simulink model "DCMachine"  (R2025b)
settings: Solver=FixedStepAuto  StartTime=0.0  StopTime=2000  FixedStep=0.01  RelTol=1e-3
values from neighbouring files (symbols this model uses):
  beta = 0.81    [DC_Motor3.m]
  d = 0.68    [DC_Motor3.m]
  En = 600-Ra*156    (= 539.16)    [DC_Motor3.m]
  I_en = 5    [DC_Motor3.m]
  Ia_max = 156    [DC_Motor3.m]
  Jeq = m_total * (rho^2 * d^2) / 4    (= 90.6180715851)    [DC_Motor3.m]
  Ki_a = Ca.Ki    [DC_Motor3.m]
  Ki_e = Ce.Ki    [DC_Motor3.m]
  Ki_w = Cw.Ki    [DC_Motor3.m]
  Kp_a = Ca.Kp    [DC_Motor3.m]
  Kp_e = Ce.Kp    [DC_Motor3.m]
  Kp_w = Cw.Kp    [DC_Motor3.m]
  Kt = 1.06    [DC_Motor3.m]
  La = tau_a * Ra    (= 0.0039)    [DC_Motor3.m]
  Le = tau_e * Re    (= 1.2)    [DC_Motor3.m]
  m_total = m_tram + m_passengers    (= 25400)    [DC_Motor3.m]
  Omega_b = 970 * (2*pi/60)    (= 101.578162466)    [DC_Motor3.m]
  Ra = 0.39    [DC_Motor3.m]
  Re = 12    [DC_Motor3.m]
  rho = 13/74    (= 0.175675675676)    [DC_Motor3.m]
  V_max = 42 * 1000/3600    (= 11.6666666667)    [DC_Motor3.m]
  V_r = Omega_b * rho * d/2    (= 6.06723619054)    [DC_Motor3.m]
libraries: slpidlib x3, simulink x1
settings Model: Creator=ASUS  LastModifiedBy=sanaz

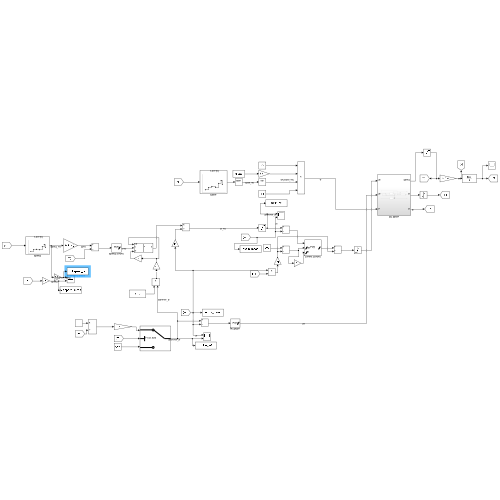
[thumbnail: Simulink's stored preview of the top-level diagram]
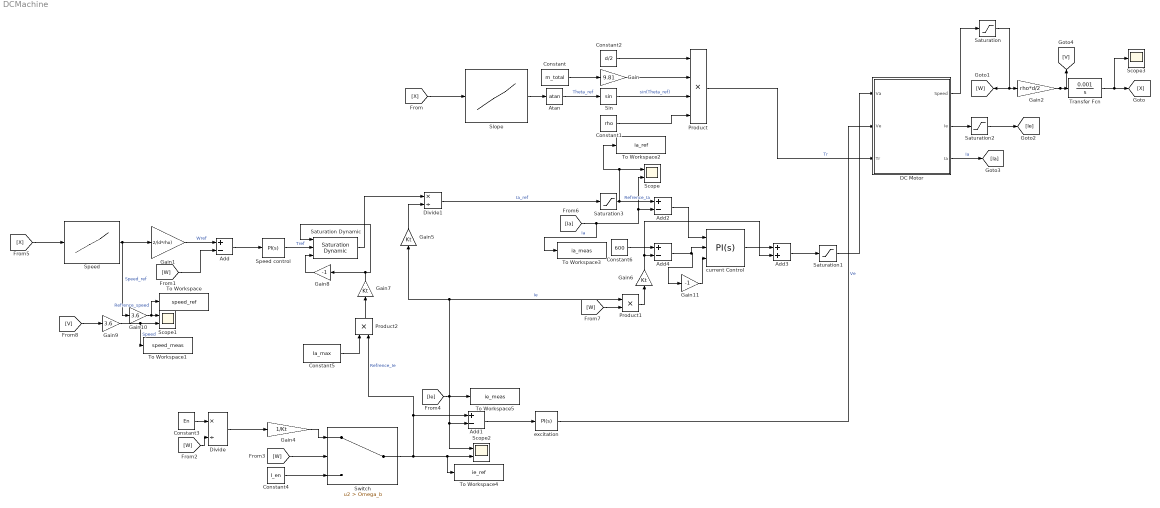
== system DCMachine ==
  Add{,1..2,4} (4 alike) : Sum  Inputs=+-
  Add3 : Sum
  Atan : Trigonometry  Operator=atan
  Constant : Constant  Value=m_total
  Constant1 : Constant  Value=rho
  Constant2 : Constant  Value=d/2
  Constant3 : Constant  Value=En
  Constant4 : Constant  Value=I_en
  Constant5 : Constant  Value=Ia_max
  Constant6 : Constant  Value=600
  DC Motor : Subsystem
  Divide : Product  Inputs=*/
  Divide1 : Product  Inputs=*/
  Gain : Gain  Gain=9.81
  Gain1 : Gain  Gain=2/(d*rho)
  Gain10 : Gain  Gain=3.6
  Gain11 : Gain  Gain=-1
  Gain2 : Gain  Gain=rho*d/2
  Gain4 : Gain  Gain=1/Kt
  Gain5 : Gain  Gain=Kt
  Gain6 : Gain  Gain=Kt
  Gain7 : Gain  Gain=Kt
  Gain8 : Gain  Gain=-1
  Gain9 : Gain  Gain=3.6
  Product : Product  Inputs=4
  Product1 : Product
  Product2 : Product
  Saturation : Saturate  UpperLimit=V_max/ (rho*d/2)  LowerLimit=-V_max/ (rho*d/2)
  Saturation Dynamic : simulink/Discontinuities/Saturation Dynamic  OutMin=[]  OutMax=[]  OutDataTypeStr=Inherit: Same as second input  OutDataType=fixdt(1, 16)  OutScaling=2^-10  DoSatur=off
  Saturation1 : Saturate  UpperLimit=600  LowerLimit=-600
  Saturation2 : Saturate  UpperLimit=inf  LowerLimit=0.0001
  Saturation3 : Saturate  UpperLimit=156  LowerLimit=-156
  Scope : Scope  NumInputPorts=2
      settings: ActiveDisplayYMinimum=-728.14495433164473  ActiveDisplayYMaximum=771.63756119337165
  Scope1 : Scope  NumInputPorts=2
      settings: ActiveDisplayYMinimum=-24.946598374660528  ActiveDisplayYMaximum=27.001405969121826
  Scope2 : Scope  NumInputPorts=2
      settings: ActiveDisplayYMinimum=-1.1065409547729188  ActiveDisplayYMaximum=6.7298853808900017  DataLoggingVariableName=ScopeData2
  Scope3 : Scope
      settings: ActiveDisplayYMinimum=-2.2097734184935658  ActiveDisplayYMaximum=19.887960766442095  DataLoggingVariableName=ScopeData3
  Sin : Trigonometry
  Slope : Lookup_n-D  NumberOfTableDimensions=1  LookupTableObject=''  BreakpointsForDimension1=[0, 1, 3, 4, 6, 8, 9, 10,10.1]  BreakpointsForDimension2=[1:2]  BreakpointsForDimension3=[5, 7]  BreakpointsForDimension1FirstPoint=10  BreakpointsForDimension2FirstPoint=10  BreakpointsForDimension1Spacing=12  BreakpointsForDimension2Spacing=12  Table=[0,0,0.05,0,0,-0.05,0,0,0]  InterpMethod=Flat  DiagnosticForOutOfRangeInput=Warning  InternalRulePriority=Speed  RndMeth=Simplest
  Speed : Lookup_n-D  NumberOfTableDimensions=1  BreakpointsForDimension1=[0, 1, 3, 4, 6, 8, 9, 10]  Table=[V_r/2,V_r,V_r,V_max,V_r,V_r,V_r/2,0]  InterpMethod=Flat  InternalRulePriority=Speed  RndMeth=Simplest
  Speed control : slpidlib/PID Controller  Controller=PI  Form=Parallel  TimeDomain=Continuous-time  UseExternalTs=off  SampleTime=-1  IntegratorMethod=Forward Euler  FilterMethod=Forward Euler  ControllerParametersSource=internal  P=Kp_w  I=Ki_w  UseKiTs=off  D=0  UseExternalDerivativeSource=off  N=100  UseFilter=on  TunerSelectOption=Transfer Function Based (PID Tuner App)  InitialConditionSource=internal  InitialConditionForIntegrator=0  InitialConditionForFilter=0  DifferentiatorICPrevScaledInput=0  ExternalReset=none  TrackingMode=off  Kt=1  LimitOutput=on  SatLimitsSource=internal  UpperSaturationLimit=827  LowerSaturationLimit=-827  LinearizeAsGain=on  AntiWindupMode=back-calculation  Kb=Ki_w/Kp_w  LimitIntegrator=on  UpperIntegratorSaturationLimit=inf  LowerIntegratorSaturationLimit=-inf  POutMin=[]  POutMax=[]  IOutMin=[]  IOutMax=[]  DOutMin=[]  DOutMax=[]  NOutMin=[]  NOutMax=[]  SumOutMin=[]  SumOutMax=[]  SaturationOutMin=[]  SaturationOutMax=[]  PParamMin=[]  PParamMax=[]  IParamMin=[]  IParamMax=[]  DParamMin=[]  DParamMax=[]  NParamMin=[]  NParamMax=[]  KbParamMin=[]  KbParamMax=[]  KtParamMin=[]  KtParamMax=[]  KbOutMin=[]  KbOutMax=[]  KtOutMin=[]  KtOutMax=[]  IntegratorOutMin=[]  IntegratorOutMax=[]  FilterOutMin=[]  FilterOutMax=[]  SumI1OutMin=[]  SumI1OutMax=[]  SumI2OutMin=[]  SumI2OutMax=[]  SumI3OutMin=[]  SumI3OutMax=[]  SumI4OutMin=[]  SumI4OutMax=[]  SumDOutMin=[]  SumDOutMax=[]  DifferentiatorOutMin=[]  DifferentiatorOutMax=[]  FilterDiffOutCoefMin=[]  FilterDiffOutCoefMax=[]  ReciprocalOutMin=[]  ReciprocalOutMax=[]  SumDenOutMin=[]  SumDenOutMax=[]  SumNumOutMin=[]  SumNumOutMax=[]  DivideOutMin=[]  DivideOutMax=[]  UdiffTsProdOutMin=[]  UdiffTsProdOutMax=[]  NTsProdOutMin=[]  NTsProdOutMax=[]  UintegralTsProdOutMin=[]  UintegralTsProdOutMax=[]  UngainTsProdOutMin=[]  UngainTsProdOutMax=[]  ClampingZeroOutDataTypeStr=Inherit: Inherit via back propagation  ClampingZeroOutMin=[]  ClampingZeroOutMax=[]  FilterDenConstantOutDataTypeStr=Inherit: Inherit via back propagation  FilterDenConstantOutMin=[]  FilterDenConstantOutMax=[]  PCopyOutDataTypeStr=Inherit: Inherit via back propagation  PCopyOutMin=[]  PCopyOutMax=[]  NCopyOutDataTypeStr=Inherit: Inherit via back propagation  NCopyOutMin=[]  NCopyOutMax=[]  IntegratorContinuousStateAttributes=''  IntegratorStateMustResolveToSignalObject=off  IntegratorRTWStateStorageClass=Auto  FilterContinuousStateAttributes=''  FilterStateMustResolveToSignalObject=off  FilterRTWStateStorageClass=Auto  ParallelPVariant=InternalParameters  IdealPVariant=Disabled  IVariant=InternalParameters  DVariant=Disabled  IntegratorVariant=Continuous  SatVariant=Enabled  AWVariant=BackCalculation  PCopyVariant=Disabled  TRVariant=Disabled  FdbkBlocksVariant=Forward  IdealPFdbkVariant=Disabled  SatFdbkVariant=Disabled  DerivativeFilterVariant=Disabled  NVariant=Disabled  NCopyVariant=Disabled_SignalSpec  FilterICVariant=Disabled  IntegratorICVariant=InternalICs  ExternalResetVariant=Disabled  TRSumVariant=Passthrough  SumFdbkVariant=Disabled  SumVariant=Sum_PI  TsampFilterVariant=InternalTs  TsampNgainVariant=Passthrough  TsampIntegralVariant=Disabled_SignalSpec  ExternalSaturationOutDataTypeStr=Inherit: Same as second input  DerivativeSourceVariant=Disabled  PreIntVariant=InternalPreInt
  Switch : Switch  Criteria=u2 > Threshold  Threshold=Omega_b  SaturateOnIntegerOverflow=off  InputSameDT=off
  To Workspace : ToWorkspace  VariableName=speed_ref  SaveFormat=Timeseries  SampleTime=-1
  To Workspace1 : ToWorkspace  VariableName=speed_meas  SaveFormat=Timeseries  SampleTime=-1
  To Workspace2 : ToWorkspace  VariableName=ia_ref  SaveFormat=Timeseries  SampleTime=-1
  To Workspace3 : ToWorkspace  VariableName=ia_meas  SaveFormat=Timeseries  SampleTime=-1
  To Workspace4 : ToWorkspace  VariableName=ie_ref  SaveFormat=Timeseries  SampleTime=-1
  To Workspace5 : ToWorkspace  VariableName=ie_meas  SaveFormat=Timeseries  SampleTime=-1
  Transfer Fcn : TransferFcn  Numerator=[0.001]  Denominator=[1 0]
  current Control : slpidlib/PID Controller  Controller=PI  Form=Parallel  TimeDomain=Continuous-time  UseExternalTs=off  SampleTime=-1  IntegratorMethod=Forward Euler  FilterMethod=Forward Euler  ControllerParametersSource=internal  P=Kp_a  I=Ki_a  UseKiTs=off  D=0  UseExternalDerivativeSource=off  N=100  UseFilter=on  TunerSelectOption=Transfer Function Based (PID Tuner App)  InitialConditionSource=internal  InitialConditionForIntegrator=0  InitialConditionForFilter=0  DifferentiatorICPrevScaledInput=0  ExternalReset=none  TrackingMode=off  Kt=1  LimitOutput=on  SatLimitsSource=external  UpperSaturationLimit=inf  LowerSaturationLimit=-inf  LinearizeAsGain=on  AntiWindupMode=back-calculation  Kb=Ki_a/Kp_a  LimitIntegrator=off  UpperIntegratorSaturationLimit=inf  LowerIntegratorSaturationLimit=-inf  POutMin=[]  POutMax=[]  IOutMin=[]  IOutMax=[]  DOutMin=[]  DOutMax=[]  NOutMin=[]  NOutMax=[]  SumOutMin=[]  SumOutMax=[]  SaturationOutMin=[]  SaturationOutMax=[]  PParamMin=[]  PParamMax=[]  IParamMin=[]  IParamMax=[]  DParamMin=[]  DParamMax=[]  NParamMin=[]  NParamMax=[]  KbParamMin=[]  KbParamMax=[]  KtParamMin=[]  KtParamMax=[]  KbOutMin=[]  KbOutMax=[]  KtOutMin=[]  KtOutMax=[]  IntegratorOutMin=[]  IntegratorOutMax=[]  FilterOutMin=[]  FilterOutMax=[]  SumI1OutMin=[]  SumI1OutMax=[]  SumI2OutMin=[]  SumI2OutMax=[]  SumI3OutMin=[]  SumI3OutMax=[]  SumI4OutMin=[]  SumI4OutMax=[]  SumDOutMin=[]  SumDOutMax=[]  DifferentiatorOutMin=[]  DifferentiatorOutMax=[]  FilterDiffOutCoefMin=[]  FilterDiffOutCoefMax=[]  ReciprocalOutMin=[]  ReciprocalOutMax=[]  SumDenOutMin=[]  SumDenOutMax=[]  SumNumOutMin=[]  SumNumOutMax=[]  DivideOutMin=[]  DivideOutMax=[]  UdiffTsProdOutMin=[]  UdiffTsProdOutMax=[]  NTsProdOutMin=[]  NTsProdOutMax=[]  UintegralTsProdOutMin=[]  UintegralTsProdOutMax=[]  UngainTsProdOutMin=[]  UngainTsProdOutMax=[]  ClampingZeroOutDataTypeStr=Inherit: Inherit via back propagation  ClampingZeroOutMin=[]  ClampingZeroOutMax=[]  FilterDenConstantOutDataTypeStr=Inherit: Inherit via back propagation  FilterDenConstantOutMin=[]  FilterDenConstantOutMax=[]  PCopyOutDataTypeStr=Inherit: Inherit via back propagation  PCopyOutMin=[]  PCopyOutMax=[]  NCopyOutDataTypeStr=Inherit: Inherit via back propagation  NCopyOutMin=[]  NCopyOutMax=[]  IntegratorContinuousStateAttributes=''  IntegratorStateMustResolveToSignalObject=off  IntegratorRTWStateStorageClass=Auto  FilterContinuousStateAttributes=''  FilterStateMustResolveToSignalObject=off  FilterRTWStateStorageClass=Auto  ParallelPVariant=InternalParameters  IdealPVariant=Disabled  IVariant=InternalParameters  DVariant=Disabled  IntegratorVariant=Continuous  SatVariant=External  AWVariant=BackCalculation  PCopyVariant=Disabled  TRVariant=Disabled  FdbkBlocksVariant=Forward  IdealPFdbkVariant=Disabled  SatFdbkVariant=Disabled  DerivativeFilterVariant=Disabled  NVariant=Disabled  NCopyVariant=Disabled_SignalSpec  FilterICVariant=Disabled  IntegratorICVariant=InternalICs  ExternalResetVariant=Disabled  TRSumVariant=Passthrough  SumFdbkVariant=Disabled  SumVariant=Sum_PI  TsampFilterVariant=InternalTs  TsampNgainVariant=Passthrough  TsampIntegralVariant=Disabled_SignalSpec  ExternalSaturationOutDataTypeStr=Inherit: Same as second input  DerivativeSourceVariant=Disabled  PreIntVariant=InternalPreInt
  excitation : slpidlib/PID Controller  Controller=PI  Form=Parallel  TimeDomain=Continuous-time  UseExternalTs=off  SampleTime=-1  IntegratorMethod=Forward Euler  FilterMethod=Forward Euler  ControllerParametersSource=internal  P=Kp_e  I=Ki_e  UseKiTs=off  D=0  UseExternalDerivativeSource=off  N=100  UseFilter=on  TunerSelectOption=Transfer Function Based (PID Tuner App)  InitialConditionSource=internal  InitialConditionForIntegrator=0  InitialConditionForFilter=0  DifferentiatorICPrevScaledInput=0  ExternalReset=none  TrackingMode=off  Kt=1  LimitOutput=on  SatLimitsSource=internal  UpperSaturationLimit=60  LowerSaturationLimit=0  LinearizeAsGain=on  AntiWindupMode=back-calculation  Kb=Ki_e/Kp_e  LimitIntegrator=off  UpperIntegratorSaturationLimit=inf  LowerIntegratorSaturationLimit=-inf  POutMin=[]  POutMax=[]  IOutMin=[]  IOutMax=[]  DOutMin=[]  DOutMax=[]  NOutMin=[]  NOutMax=[]  SumOutMin=[]  SumOutMax=[]  SaturationOutMin=[]  SaturationOutMax=[]  PParamMin=[]  PParamMax=[]  IParamMin=[]  IParamMax=[]  DParamMin=[]  DParamMax=[]  NParamMin=[]  NParamMax=[]  KbParamMin=[]  KbParamMax=[]  KtParamMin=[]  KtParamMax=[]  KbOutMin=[]  KbOutMax=[]  KtOutMin=[]  KtOutMax=[]  IntegratorOutMin=[]  IntegratorOutMax=[]  FilterOutMin=[]  FilterOutMax=[]  SumI1OutMin=[]  SumI1OutMax=[]  SumI2OutMin=[]  SumI2OutMax=[]  SumI3OutMin=[]  SumI3OutMax=[]  SumI4OutMin=[]  SumI4OutMax=[]  SumDOutMin=[]  SumDOutMax=[]  DifferentiatorOutMin=[]  DifferentiatorOutMax=[]  FilterDiffOutCoefMin=[]  FilterDiffOutCoefMax=[]  ReciprocalOutMin=[]  ReciprocalOutMax=[]  SumDenOutMin=[]  SumDenOutMax=[]  SumNumOutMin=[]  SumNumOutMax=[]  DivideOutMin=[]  DivideOutMax=[]  UdiffTsProdOutMin=[]  UdiffTsProdOutMax=[]  NTsProdOutMin=[]  NTsProdOutMax=[]  UintegralTsProdOutMin=[]  UintegralTsProdOutMax=[]  UngainTsProdOutMin=[]  UngainTsProdOutMax=[]  ClampingZeroOutDataTypeStr=Inherit: Inherit via back propagation  ClampingZeroOutMin=[]  ClampingZeroOutMax=[]  FilterDenConstantOutDataTypeStr=Inherit: Inherit via back propagation  FilterDenConstantOutMin=[]  FilterDenConstantOutMax=[]  PCopyOutDataTypeStr=Inherit: Inherit via back propagation  PCopyOutMin=[]  PCopyOutMax=[]  NCopyOutDataTypeStr=Inherit: Inherit via back propagation  NCopyOutMin=[]  NCopyOutMax=[]  IntegratorContinuousStateAttributes=''  IntegratorStateMustResolveToSignalObject=off  IntegratorRTWStateStorageClass=Auto  FilterContinuousStateAttributes=''  FilterStateMustResolveToSignalObject=off  FilterRTWStateStorageClass=Auto  ParallelPVariant=InternalParameters  IdealPVariant=Disabled  IVariant=InternalParameters  DVariant=Disabled  IntegratorVariant=Continuous  SatVariant=Enabled  AWVariant=BackCalculation  PCopyVariant=Disabled  TRVariant=Disabled  FdbkBlocksVariant=Forward  IdealPFdbkVariant=Disabled  SatFdbkVariant=Disabled  DerivativeFilterVariant=Disabled  NVariant=Disabled  NCopyVariant=Disabled_SignalSpec  FilterICVariant=Disabled  IntegratorICVariant=InternalICs  ExternalResetVariant=Disabled  TRSumVariant=Passthrough  SumFdbkVariant=Disabled  SumVariant=Sum_PI  TsampFilterVariant=InternalTs  TsampNgainVariant=Passthrough  TsampIntegralVariant=Disabled_SignalSpec  ExternalSaturationOutDataTypeStr=Inherit: Same as second input  DerivativeSourceVariant=Disabled  PreIntVariant=InternalPreInt
  wires:
  Slope/1 -> Atan/1
  Atan/1 -> Sin/1  "Theta_ref"
  Constant/1 -> Gain/1
  Gain/1 -> Product/2
  Sin/1 -> Product/3  "sin(Theta_ref)"
  Constant1/1 -> Product/4
  Speed/1 -> Gain10/1, Gain1/1  "Speed_ref"
  Gain1/1 -> Add/1  "Wref"
  Product/1 -> DC Motor/3(Tr)  "Tr"
  DC Motor/1(Speed) -> Saturation/1
  Saturation/1 -> [W], Gain2/1
  Gain2/1 -> [V], Transfer Fcn/1
  Transfer Fcn/1 -> Scope3/1, [X]
  [X] -> Slope/1
  [W] -> Add/2
  Constant3/1 -> Divide/1
  [W] -> Divide/2
  [W] -> Switch/2
  Constant4/1 -> Switch/3
  Divide/1 -> Gain4/1
  Gain4/1 -> Switch/1
  Switch/1 -> Product2/2, Add1/1, To Workspace4/1, Scope2/2  "Refrence_Ie"
  [Ie] -> To Workspace5/1, Product1/1, Gain5/1, Scope2/1, Add1/2  "Ie"
  Add1/1 -> excitation/1
  excitation/1 -> DC Motor/2(Ve)  "Ve"
  [X] -> Speed/1
  Add/1 -> Speed control/1
  Gain5/1 -> Divide1/2
  Divide1/1 -> Saturation3/1  "Ia_ref"
  DC Motor/3(Ia) -> [Ia]  "Ia"
  [Ia] -> To Workspace3/1, Add2/2, Scope/2  "Ia"
  Add2/1 -> current Control/1
  current Control/1 -> Add3/1
  Gain6/1 -> Add4/2, Add3/2
  Product1/1 -> Gain6/1
  [W] -> Product1/2
  Add3/1 -> Saturation1/1
  Saturation1/1 -> DC Motor/1(Va)
  Speed control/1 -> Saturation Dynamic/2  "Tref"
  Product2/1 -> Gain7/1
  Constant5/1 -> Product2/1
  Gain7/1 -> Saturation Dynamic/1, Gain8/1
  Gain8/1 -> Saturation Dynamic/3
  Saturation Dynamic/1 -> Divide1/1
  [V] -> Gain9/1
  Gain9/1 -> To Workspace1/1, Scope1/2  "Speed"
  Gain10/1 -> To Workspace/1, Scope1/1  "Refrence_speed"
  Constant6/1 -> Add4/1
  Add4/1 -> current Control/2, Gain11/1
  Gain11/1 -> current Control/3
  DC Motor/2(Ie) -> Saturation2/1
  Saturation2/1 -> [Ie]
  Saturation3/1 -> Scope/1, To Workspace2/1, Add2/1  "Refrence_Ia"
  Constant2/1 -> Product/1

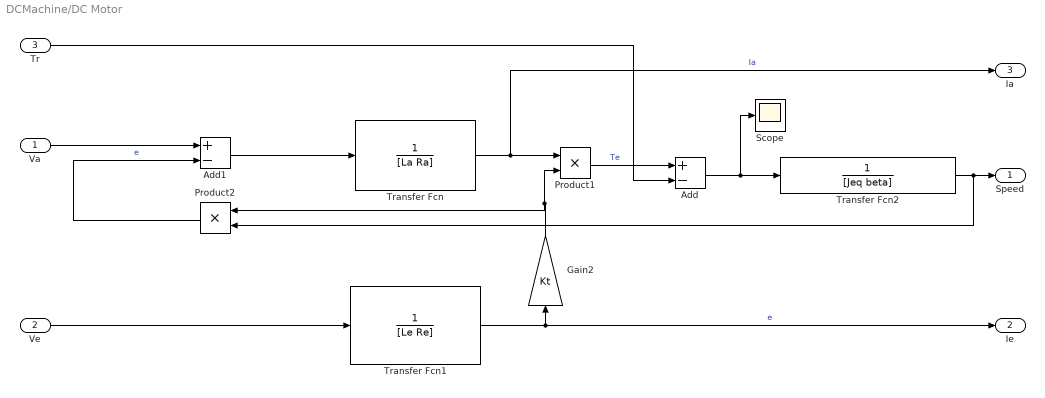
== system DCMachine/DC Motor ==
  Va : Inport
  Ve : Inport  Port=2
  Tr : Inport  Port=3
  Add : Sum  Inputs=+-
  Add1 : Sum  Inputs=+-
  Gain2 : Gain  Gain=Kt
  Product1 : Product
  Product2 : Product
  Scope : Scope
      settings: DataLoggingVariableName=ScopeData5
  Transfer Fcn : TransferFcn  Denominator=[La Ra]
  Transfer Fcn1 : TransferFcn  Denominator=[Le Re]
  Transfer Fcn2 : TransferFcn  Denominator=[Jeq beta]
  Speed : Outport
  Ie : Outport  Port=2
  Ia : Outport  Port=3
  wires:
  Transfer Fcn1/1 -> Ie/1, Gain2/1  "e"
  Va/1 -> Add1/1
  Add1/1 -> Transfer Fcn/1
  Ve/1 -> Transfer Fcn1/1
  Transfer Fcn/1 -> Ia/1, Product1/1  "Ia"
  Transfer Fcn2/1 -> Product2/2, Speed/1
  Gain2/1 -> Product2/1, Product1/2
  Product2/1 -> Add1/2  "e"
  Product1/1 -> Add/1  "Te"
  Tr/1 -> Add/2
  Add/1 -> Scope/1, Transfer Fcn2/1
